simulink model "implcmd_can_pack"  (R2026b)
settings: Solver=VariableStepAuto
undefined symbols (not defined in the file or in its folder): Ts
libraries: simulink x1, svdutilitieslib x1
settings Model: Creator=aomar  LastModifiedBy=aomar

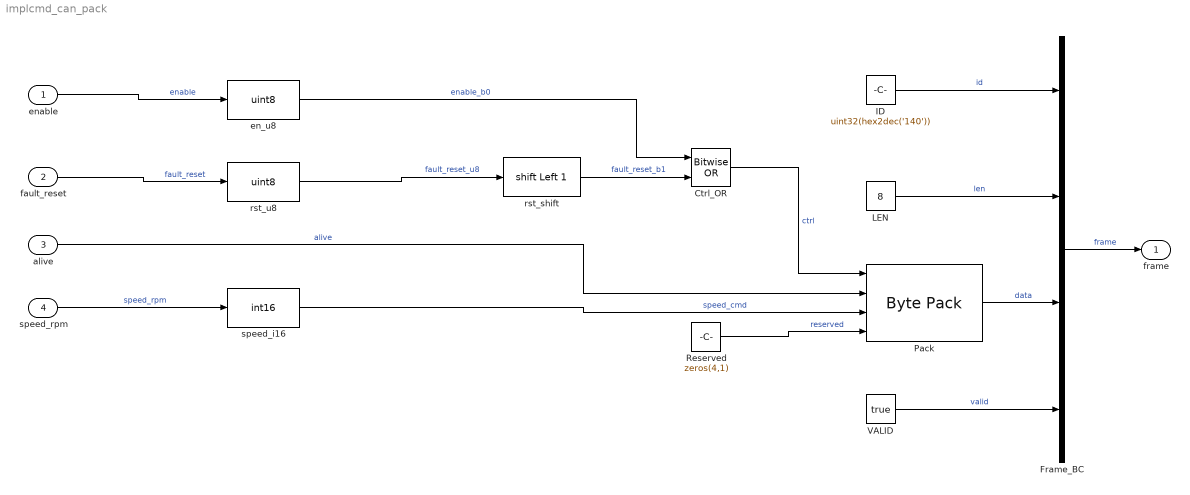
== system implcmd_can_pack ==
  enable : Inport  OutDataTypeStr=boolean  PortDimensions=1  SampleTime=Ts.can_slow
  fault_reset : Inport  Port=2  OutDataTypeStr=boolean  PortDimensions=1  SampleTime=Ts.can_slow
  alive : Inport  Port=3  OutDataTypeStr=uint8  PortDimensions=1  SampleTime=Ts.can_slow
  speed_rpm : Inport  Port=4  OutDataTypeStr=single  PortDimensions=1  SampleTime=Ts.can_slow
  Ctrl_OR : simulink/Logic and Bit Operations/Bitwise Operator  logicop=OR  UseBitMask=off  NumInputPorts=2  BitMask=bin2dec('11011001')  BitMaskRealWorld=Stored Integer
  Frame_BC : BusCreator  Inputs=4  OutDataTypeStr=Bus: Bus_CanFrame8  NonVirtualBus=on
      settings: InheritFromInputs=off
  ID : Constant  Value=uint32(hex2dec('140'))  OutDataTypeStr=uint32  SampleTime=Ts.can_slow
  LEN : Constant  Value=8  OutDataTypeStr=uint8  SampleTime=Ts.can_slow
  Pack : svdutilitieslib/Byte Pack  maskPackedDataType=uint8  datatypes={'uint8','uint8','int16','uint8'}  byteAlign=1  blockPlatform=arduinoert
      settings: LibrarySourceBlock=mcblib/Signal Management/Byte Pack
  Reserved : Constant  Value=zeros(4,1)  OutDataTypeStr=uint8  SampleTime=Ts.can_slow
  VALID : Constant  Value=true  OutDataTypeStr=boolean  SampleTime=Ts.can_slow
  en_u8 : DataTypeConversion  OutDataTypeStr=uint8  RndMeth=Nearest
  rst_shift : ArithShift  BitShiftNumber=1  BitShiftDirection=Left
  rst_u8 : DataTypeConversion  OutDataTypeStr=uint8  RndMeth=Nearest
  speed_i16 : DataTypeConversion  OutDataTypeStr=int16  RndMeth=Nearest
  frame : Outport  OutDataTypeStr=Bus: Bus_CanFrame8
  wires:
  enable/1 -> en_u8/1  "enable"
  fault_reset/1 -> rst_u8/1  "fault_reset"
  alive/1 -> Pack/2  "alive"
  speed_rpm/1 -> speed_i16/1  "speed_rpm"
  en_u8/1 -> Ctrl_OR/1  "enable_b0"
  rst_u8/1 -> rst_shift/1  "fault_reset_u8"
  speed_i16/1 -> Pack/3  "speed_cmd"
  rst_shift/1 -> Ctrl_OR/2  "fault_reset_b1"
  Reserved/1 -> Pack/4  "reserved"
  Ctrl_OR/1 -> Pack/1  "ctrl"
  ID/1 -> Frame_BC/1  "id"
  LEN/1 -> Frame_BC/2  "len"
  VALID/1 -> Frame_BC/4  "valid"
  Pack/1 -> Frame_BC/3  "data"
  Frame_BC/1 -> frame/1  "frame"
